simulink model "xygraph"  (Simulink 5.0)
settings: Solver=ode45  StartTime=0.0  StopTime=10.0  RelTol=1e-3
undefined symbols (not defined in the file or in its folder): sigbuilder_block
settings Model: Creator=mcarroll  LastModifiedBy=mcarroll  ExtModeAutoUpdateStatusClock=off

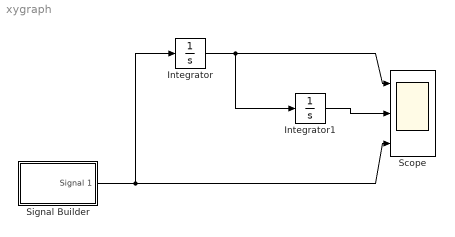
== system xygraph ==
  Integrator : Integrator
  Integrator1 : Integrator
  Scope : Scope  NumInputPorts=3
      settings: YMin=-5~-5~-5  YMax=5~5~5
  Signal Builder : Subsystem  Tag=STV Subsys  LoadFcn=sigbuilder_block('open',[68 101.6 520 400 ]);  StartFcn=sigbuilder_block('start');  StopFcn=sigbuilder_block('stop');  ClipboardFcn=sigbuilder_block('clipboard');  mask(Sigbuilder block){}
      mask help: Sigbuilder GUI
      mask init:
      | if ~strcmp(get_param(bdroot(gcb),'SimulationStatus'),'stopped') tuvar = sigbuilder_block('maskInit'); end
      settings: CopyFcn=sigbuilder_block('copy');  DeleteFcn=sigbuilder_block('delete');  ModelCloseFcn=sigbuilder_block('modelClose');  PreSaveFcn=sigbuilder_block('preSave');  NameChangeFcn=sigbuilder_block('namechange');  OpenFcn=sigbuilder_block('open',[68 101.6 520 400 ]);  CloseFcn=sigbuilder_block('close');
      mask Display: plot(0,0,100,100,[10,10,40,40,10],[80,20,20,80,80],[40,10],[50,50], [40,27,10],[65,72,56],[40,25,25,10],[28,28,43,43]);
  wires:
  Signal Builder/1(Signal 1) -> Integrator/1, Scope/3
  Integrator/1 -> Scope/1, Integrator1/1
  Integrator1/1 -> Scope/2

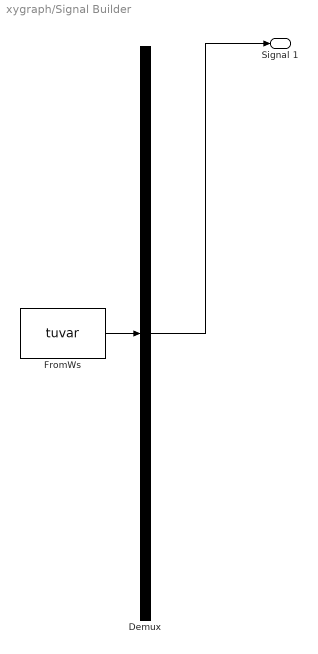
== system xygraph/Signal Builder ==
  Demux : Demux  Tag=STV Demux  Outputs=1
  FromWs : FromWorkspace  Tag=STV FromWs  VariableName=tuvar  SampleTime=0  SigBuilderData=DataTag0
      SigBuilderData=|
      | channels.label = 'Signal 1'
      | channels.allXData = {[0 4 4 6.04 6.04 10]}
      | channels.allYData = {[0 0.19 0.5 -0.49 0 0]}
      | dataSet.timeRange = [0 10]
      | dataSet.name = 'Group 1'
  Signal 1 : Outport  Tag=STV Outport
  wires:
  Demux/1 -> Signal 1/1
  FromWs/1 -> Demux/1
